simulink model "FuzzyPID_Temperature_Control"  (R2024a)
settings: Solver=VariableStepAuto  StartTime=0.0  StopTime=600  RelTol=1e-3
libraries: fuzblock x1, slpidlib x1
settings Model: Creator=ffgxf  LastModifiedBy=ffgxf

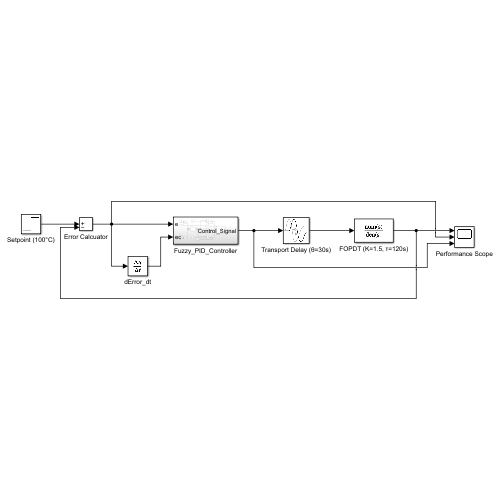
[thumbnail: Simulink's stored preview of the top-level diagram]
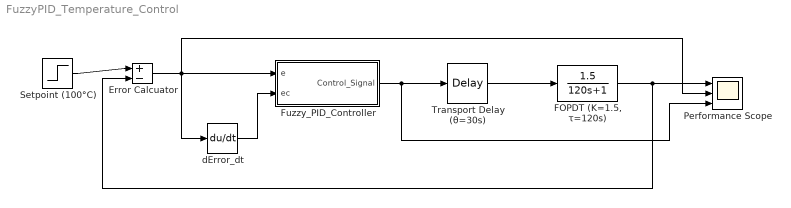
== system FuzzyPID_Temperature_Control ==
  Error Calcuator : Sum  Inputs=|+-
  "FOPDT (K=1.5, τ=120s)" : TransferFcn  Numerator=[1.5]  Denominator=[120 1]
  Fuzzy_PID_Controller : Subsystem
  Performance Scope : Scope  NumInputPorts=3
  Setpoint (100°C) : Step  Time=0  After=100  SampleTime=0.5
  Transport Delay (θ=30s) : TransportDelay  DelayTime=30  FixedBuffer=on
  dError_dt : Derivative
  wires:
  Setpoint (100°C)/1 -> Error Calcuator/1
  Error Calcuator/1 -> Fuzzy_PID_Controller/1(e), dError_dt/1, Performance Scope/2
  dError_dt/1 -> Fuzzy_PID_Controller/2(ec)
  Fuzzy_PID_Controller/1(Control_Signal) -> Transport Delay (θ=30s)/1, Performance Scope/3
  Transport Delay (θ=30s)/1 -> "FOPDT (K=1.5, τ=120s)"/1
  "FOPDT (K=1.5, τ=120s)"/1 -> Performance Scope/1, Error Calcuator/2

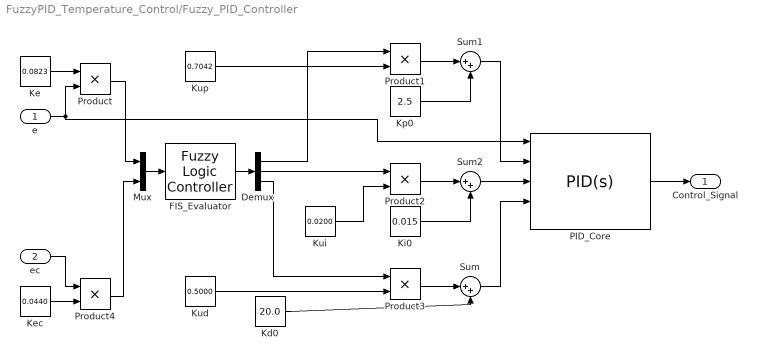
== system FuzzyPID_Temperature_Control/Fuzzy_PID_Controller ==
  e : Inport
  ec : Inport  Port=2
  Demux : Demux  Outputs=3
  FIS_Evaluator : fuzblock/Fuzzy Logic  Controller  FIS=fuzzy_pid_controller  OutputSampleNumber=101  DataType=double  FuzzifiedInputs=off  RuleFiringStrengths=off  RuleOutputs=off  AggregatedOutputs=off  SimulateUsing=Interpreted execution  OutOfRangeInputValueMessage=warning  NoRuleFiredMessage=warning  EmptyOutputFuzzySetMessage=warning
  Kd0 : Constant  Value=20.0
  Ke : Constant  Value=0.0823
  Kec : Constant  Value=0.0440
  Ki0 : Constant  Value=0.015
  Kp0 : Constant  Value=2.5
  Kud : Constant  Value=0.5000
  Kui : Constant  Value=0.0200
  Kup : Constant  Value=0.7042
  Mux : Mux  Inputs=2
  PID_Core : slpidlib/PID Controller  Controller=PID  Form=Parallel  TimeDomain=Continuous-time  UseExternalTs=off  SampleTime=-1  IntegratorMethod=Forward Euler  FilterMethod=Forward Euler  ControllerParametersSource=external  P=1  I=1  UseKiTs=off  D=0  UseExternalDerivativeSource=off  N=100  UseFilter=on  TunerSelectOption=Transfer Function Based (PID Tuner App)  InitialConditionSource=internal  InitialConditionForIntegrator=0  InitialConditionForFilter=0  DifferentiatorICPrevScaledInput=0  ExternalReset=none  TrackingMode=off  Kt=1  LimitOutput=on  SatLimitsSource=internal  UpperSaturationLimit=150  LowerSaturationLimit=0  LinearizeAsGain=on  AntiWindupMode=none  Kb=1  LimitIntegrator=off  UpperIntegratorSaturationLimit=inf  LowerIntegratorSaturationLimit=-inf  POutMin=[]  POutMax=[]  IOutMin=[]  IOutMax=[]  DOutMin=[]  DOutMax=[]  NOutMin=[]  NOutMax=[]  SumOutMin=[]  SumOutMax=[]  SaturationOutMin=[]  SaturationOutMax=[]  PParamMin=[]  PParamMax=[]  IParamMin=[]  IParamMax=[]  DParamMin=[]  DParamMax=[]  NParamMin=[]  NParamMax=[]  KbParamMin=[]  KbParamMax=[]  KtParamMin=[]  KtParamMax=[]  KbOutMin=[]  KbOutMax=[]  KtOutMin=[]  KtOutMax=[]  IntegratorOutMin=[]  IntegratorOutMax=[]  FilterOutMin=[]  FilterOutMax=[]  SumI1OutMin=[]  SumI1OutMax=[]  SumI2OutMin=[]  SumI2OutMax=[]  SumI3OutMin=[]  SumI3OutMax=[]  SumI4OutMin=[]  SumI4OutMax=[]  SumDOutMin=[]  SumDOutMax=[]  DifferentiatorOutMin=[]  DifferentiatorOutMax=[]  FilterDiffOutCoefMin=[]  FilterDiffOutCoefMax=[]  ReciprocalOutMin=[]  ReciprocalOutMax=[]  SumDenOutMin=[]  SumDenOutMax=[]  SumNumOutMin=[]  SumNumOutMax=[]  DivideOutMin=[]  DivideOutMax=[]  UdiffTsProdOutMin=[]  UdiffTsProdOutMax=[]  NTsProdOutMin=[]  NTsProdOutMax=[]  UintegralTsProdOutMin=[]  UintegralTsProdOutMax=[]  UngainTsProdOutMin=[]  UngainTsProdOutMax=[]  ClampingZeroOutDataTypeStr=Inherit: Inherit via back propagation  ClampingZeroOutMin=[]  ClampingZeroOutMax=[]  FilterDenConstantOutDataTypeStr=Inherit: Inherit via back propagation  FilterDenConstantOutMin=[]  FilterDenConstantOutMax=[]  PCopyOutDataTypeStr=Inherit: Inherit via back propagation  PCopyOutMin=[]  PCopyOutMax=[]  NCopyOutDataTypeStr=Inherit: Inherit via back propagation  NCopyOutMin=[]  NCopyOutMax=[]  IntegratorContinuousStateAttributes=''  IntegratorStateMustResolveToSignalObject=off  IntegratorRTWStateStorageClass=Auto  FilterContinuousStateAttributes=''  FilterStateMustResolveToSignalObject=off  FilterRTWStateStorageClass=Auto  ParallelPVariant=ExternalParameters  IdealPVariant=Disabled  IVariant=ExternalParameters  DVariant=ExternalParameters  IntegratorVariant=Continuous  SatVariant=Enabled  AWVariant=Passthrough  PCopyVariant=Disabled  TRVariant=Disabled  FdbkBlocksVariant=Forward  IdealPFdbkVariant=Disabled  SatFdbkVariant=Disabled  DerivativeFilterVariant=ContFilter  NVariant=ExternalParameters  NCopyVariant=Disabled  FilterICVariant=InternalICsFilter  IntegratorICVariant=InternalICs  ExternalResetVariant=Disabled  TRSumVariant=Passthrough  SumFdbkVariant=Disabled  SumVariant=Sum_PID  TsampFilterVariant=InternalTs  TsampNgainVariant=Passthrough  TsampIntegralVariant=Disabled_SignalSpec  ExternalSaturationOutDataTypeStr=Inherit: Same as second input  DerivativeSourceVariant=ErrorSignal
  Product{,1..4} (5 alike) : Product
  Sum : Sum  Inputs=|++
  Sum1 : Sum  Inputs=|++
  Sum2 : Sum  Inputs=|++
  Control_Signal : Outport
  wires:
  Kp0/1 -> Sum1/2
  e/1 -> Product/2, PID_Core/1
  Ke/1 -> Product/1
  ec/1 -> Product4/1
  Kec/1 -> Product4/2
  Mux/1 -> FIS_Evaluator/1
  Product/1 -> Mux/1
  Product4/1 -> Mux/2
  Kup/1 -> Product1/2
  Product1/1 -> Sum1/1
  Sum1/1 -> PID_Core/2
  PID_Core/1 -> Control_Signal/1
  FIS_Evaluator/1 -> Demux/1
  Demux/1 -> Product1/1
  Demux/2 -> Product2/1
  Kui/1 -> Product2/2
  Product2/1 -> Sum2/1
  Ki0/1 -> Sum2/2
  Sum2/1 -> PID_Core/3
  Demux/3 -> Product3/1
  Kud/1 -> Product3/2
  Product3/1 -> Sum/1
  Kd0/1 -> Sum/2
  Sum/1 -> PID_Core/4
